simulink model "Simple_EV_Charger"  (R2024b)
settings: Solver=ode8  StartTime=0.0  StopTime=1.5  FixedStep=1e-6  RelTol=1e-3
undefined symbols (not defined in the file): Acid, Lead
libraries: spsDiodeLib x10, spsMosfetLib x6, spsCurrentMeasurementLib x5, spsSeriesRLCBranchLib x5, spsVoltageMeasurementLib x4, slpidlib x3, spsACVoltageSourceLib x1, spsBatteryLib x1, spsLinearTransformerLib x1, spsRMSLib x1, simulink x1, spsIdealSwitchLib x1
settings Model: Creator=SUDHAK1  LastModifiedBy=SUDHAK1

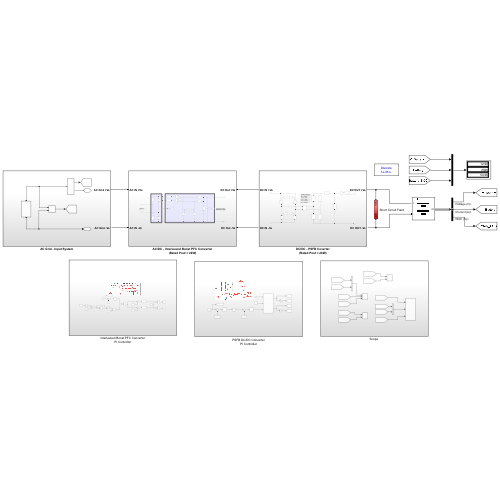
[thumbnail: Simulink's stored preview of the top-level diagram]
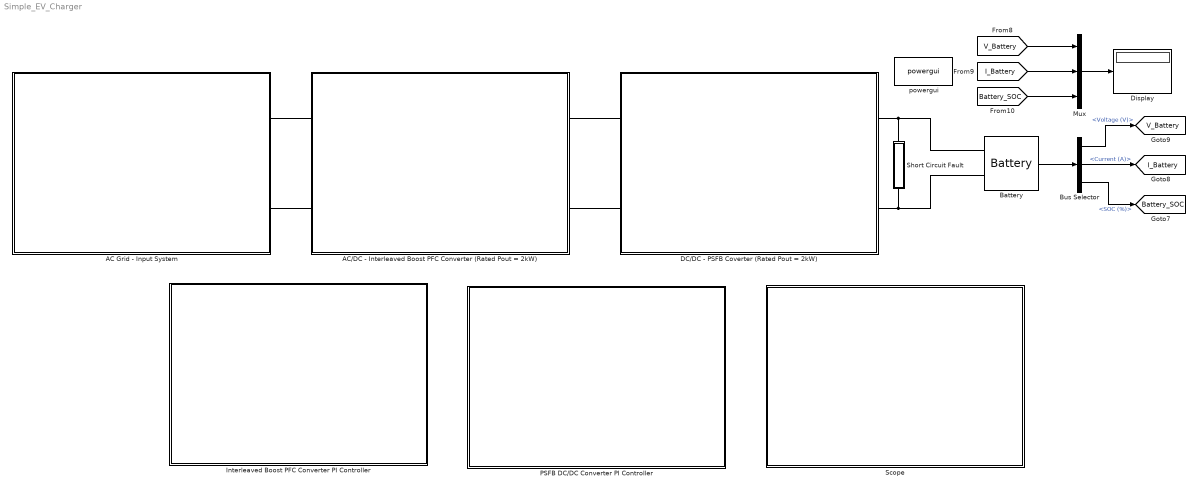
== system Simple_EV_Charger ==
  AC Grid - Input System : Subsystem
  AC/DC - Interleaved Boost PFC Converter (Rated Pout = 2kW) : Subsystem
  Battery : spsBatteryLib/Battery  BatType=Lead-Acid  NomV=48  NomQ=150  SOC=50  Batt_Tr=1  PresetModel=on  MaxQ=156.25  MinV=36  FullV=52.2632  Dis_rate=30  R=0.0032  Normal_OP=46.5417  expZone="[48.8684          0.5]"
  Bus Selector : BusSelector  OutputSignals=Voltage (V),Current (A),SOC (%)
  DC/DC - PSFB Coverter (Rated Pout = 2kW) : Subsystem
  Display : Display
  Interleaved Boost PFC Converter PI Controller : Subsystem
  Mux : Mux  Inputs=3
  PSFB DC/DC Converter PI Controller : Subsystem
  "Scope " : Subsystem
  Short Circuit Fault : Subsystem
      settings: PortSchema="{\"entries\":[{\"content\":{\"sides\":[{\"content\":{},\"type\":\"ConnectorPlacement.EquallySpacedRectSide\",\"uuid\":\"d1eece8f-50e0-4bd3-bd02-64a44f95c15f\"},{\"content\":{\"side\":\"RIGHT\"},\"type\":\"ConnectorPlacement.EquallySpacedRectSide\",\"uuid\":\"d3715762-f460-4a18-a379-b690b190937e\"},{\"content\":{\"connectorIds\":[\"LConn1\"],\"side\":\"TOP\"},\"type\":\"ConnectorPlacement.EquallySpacedRectSide\",\"uuid\":\"cdaaabb7-d644-4e36-8adb-959b7298db19\"},{\"content\":{\"connectorIds\":[\"RConn1\"],\"side\":\"BOTTOM\"},\"type\":\"ConnectorPlacement.EquallySpacedRectSide\",\"uuid\":\"a0244b95-e79a-4abc-836f-bd8cb9c3c8a7\"}]},\"type\":\"ConnectorPlacement.EquallySpacedConnector\",\"uuid\":\"f19808b0-397b-4bab-947c-d2711a911d87\"}],\"packageUris\":[\"http://schema.mathworks.com/mf0/Connector/R2020b\"],\"version\":\"1.0\"}"
  powergui : spspowerguiLib/powergui  Priority=1  SimulationMode=Discrete  SampleTime=1e-6  frequency=60  Iterations=50  frequencyindice=50  Pbase=100e6  ErrMax=1e-4  UnitsV=kV  UnitsW=MW  buscounter=0  FunctionMessages=off  echomessages=off  EnableUseOfTLC=off  CurrentSourceSwitches=off  DisableSnubberDevices=off  DisableRonSwitches=off  DisableVfSwitches=off  DisplayEquations=off  AutomaticDiscreteSolvers=off  SolverType=Tustin/Backward Euler (TBE)  Interpol=off  ExternalGateDelay=off  methode=off  Ts=100  x0status=blocks  SPID=on  SwTol=0  HookPort=off  NonlinearTolerance=1e-4  nMaxIteration=100  ContinueOnMaxIteration=off  RestoreLinks=warning  ResistiveCurrentMeasurement=off  Frange=[0:2:500]  Ylog=off  Xlog=on  ShowGrid=off  save=off  variable=ZData  structure=0  ZoomFFT=off  StartTime=0.0  cycles=1  DisplayStyle=1  fundamental=60  FreqAxis=off  MaxFrequency=1000  frequencyindicesteady=1  RmsSteady=1  display=off
  tag scope: Battery_SOC=global, I_Battery=global, V_Battery=global
  wires:
  Battery/1 -> Bus Selector/1
  Bus Selector/3 -> [Battery_SOC]  "<SOC (%)>"
  Bus Selector/2 -> [I_Battery]  "<Current (A)>"
  Bus Selector/1 -> [V_Battery]  "<Voltage (V)>"
  [V_Battery] -> Mux/1
  [I_Battery] -> Mux/2
  Mux/1 -> Display/1
  [Battery_SOC] -> Mux/3
  connections:
  AC Grid - Input System/RConn1 -- AC/DC - Interleaved Boost PFC Converter (Rated Pout = 2kW)/LConn1
  AC Grid - Input System/RConn2 -- AC/DC - Interleaved Boost PFC Converter (Rated Pout = 2kW)/LConn2
  AC/DC - Interleaved Boost PFC Converter (Rated Pout = 2kW)/RConn1 -- DC/DC - PSFB Coverter (Rated Pout = 2kW)/LConn1
  Battery/LConn1 -- DC/DC - PSFB Coverter (Rated Pout = 2kW)/RConn1 -- Short Circuit Fault/LConn1
  DC/DC - PSFB Coverter (Rated Pout = 2kW)/RConn2 -- Battery/LConn2 -- Short Circuit Fault/RConn1
  DC/DC - PSFB Coverter (Rated Pout = 2kW)/LConn2 -- AC/DC - Interleaved Boost PFC Converter (Rated Pout = 2kW)/RConn2

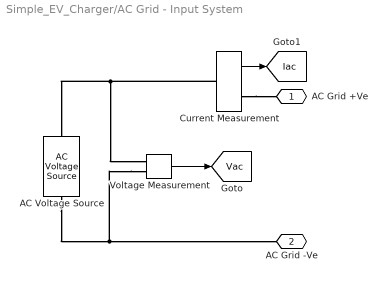
== system Simple_EV_Charger/AC Grid - Input System ==
  AC Voltage Source : spsACVoltageSourceLib/AC Voltage Source  Amplitude=230*sqrt(2)  Phase=0  Frequency=50  SampleTime=0  Measurements=None  BusType=swing  Pref=10e3  Qref=0  Qmin=-inf  Qmax=+inf
  Current Measurement : spsCurrentMeasurementLib/Current Measurement  PhasorSimulation=off  OutputType=Complex  PSBequivalent=0
  Voltage Measurement : spsVoltageMeasurementLib/Voltage Measurement  PhasorSimulation=off  OutputType=Complex  PSBequivalent=0
  AC Grid +Ve : PMIOPort  Side=Right
  AC Grid -Ve : PMIOPort  Port=2  Side=Right
  tag scope: Iac=global, Vac=global
  wires:
  Current Measurement/1 -> [Iac]
  Voltage Measurement/1 -> [Vac]
  connections:
  Voltage Measurement/LConn2 -- AC Grid -Ve/RConn1 -- AC Voltage Source/LConn1
  Current Measurement/LConn1 -- AC Voltage Source/RConn1 -- Voltage Measurement/LConn1
  Current Measurement/RConn1 -- AC Grid +Ve/RConn1

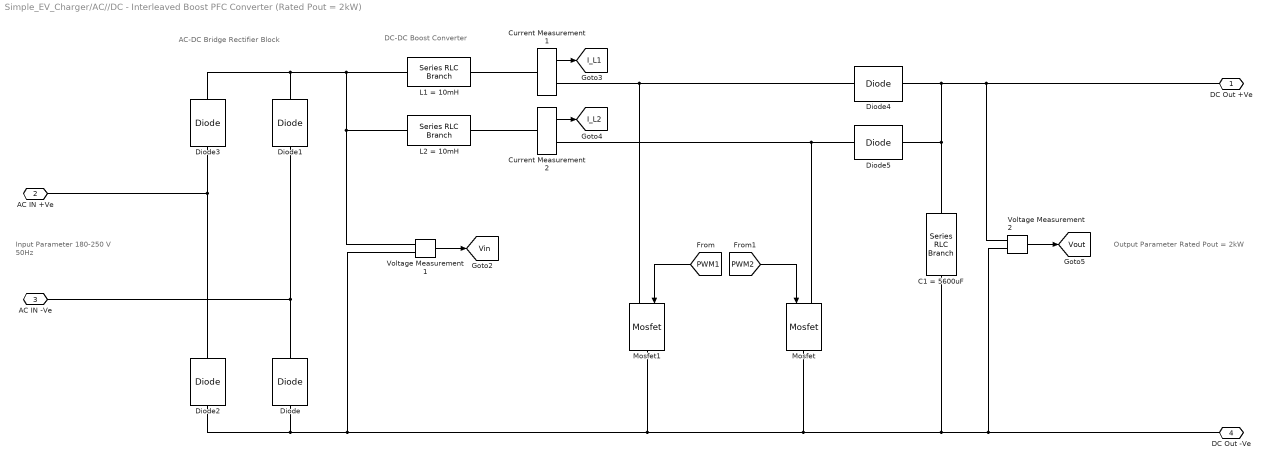
== system Simple_EV_Charger/AC//DC - Interleaved Boost PFC Converter (Rated Pout = 2kW) ==
  note: DC-DC Boost Converter
  note: AC-DC Bridge Rectifier Block
  note: Input Parameter
      | 180-250 V
      | 50Hz
  note: Output Parameter
      | Rated Pout = 2kW
  C1 = 5600uF : spsSeriesRLCBranchLib/Series RLC Branch  LConnTagsString=__new0  RConnTagsString=__new0  BranchType=RC  Resistance=0.02  Inductance=10e-3  SetiL0=off  InitialCurrent=0  Capacitance=5600e-6  Setx0=off  InitialVoltage=0  Measurements=None
  Current Measurement1 : spsCurrentMeasurementLib/Current Measurement  PhasorSimulation=off  OutputType=Complex  PSBequivalent=0
  Current Measurement2 : spsCurrentMeasurementLib/Current Measurement  PhasorSimulation=off  OutputType=Complex  PSBequivalent=0
  Diode{,1..5} (6 alike) : spsDiodeLib/Diode  Ron=1e-3  Lon=0  Vf=0.8  IC=0  UseSnubber=0  Rs=500  Cs=250e-9  Measurements=off
  L1 = 10mH : spsSeriesRLCBranchLib/Series RLC Branch  LConnTagsString=__new0  RConnTagsString=__new0  BranchType=L  Resistance=1  Inductance=10e-3  SetiL0=off  InitialCurrent=0  Capacitance=1e-6  Setx0=off  InitialVoltage=0  Measurements=None
  L2 = 10mH : spsSeriesRLCBranchLib/Series RLC Branch  LConnTagsString=__new0  RConnTagsString=__new0  BranchType=L  Resistance=1  Inductance=10e-3  SetiL0=off  InitialCurrent=0  Capacitance=1e-6  Setx0=off  InitialVoltage=0  Measurements=None
  Mosfet : spsMosfetLib/Mosfet  Ron=0.1  Lon=0  Rd=0.01  Vfd=0  IC=0  Rs=1e5  Cs=inf  Measurements=off
  Mosfet1 : spsMosfetLib/Mosfet  Ron=0.1  Lon=0  Rd=0.01  Vfd=0  IC=0  Rs=1e5  Cs=inf  Measurements=off
  Voltage Measurement1 : spsVoltageMeasurementLib/Voltage Measurement  PhasorSimulation=off  OutputType=Complex  PSBequivalent=0
  Voltage Measurement2 : spsVoltageMeasurementLib/Voltage Measurement  PhasorSimulation=off  OutputType=Complex  PSBequivalent=0
  DC Out +Ve : PMIOPort  Side=Right
  AC IN +Ve : PMIOPort  Port=2  Side=Left
  AC IN -Ve : PMIOPort  Port=3  Side=Left
  DC Out -Ve : PMIOPort  Port=4  Side=Right
  tag scope: I_L1=global, I_L2=global, Vin=global, Vout=global
  wires:
  Current Measurement2/1 -> [I_L2]
  Voltage Measurement2/1 -> [Vout]
  Current Measurement1/1 -> [I_L1]
  Voltage Measurement1/1 -> [Vin]
  [PWM1] -> Mosfet1/1
  [PWM2] -> Mosfet/1
  connections:
  Diode4/LConn1 -- Current Measurement1/RConn1 -- Mosfet1/LConn1
  Diode5/RConn1 -- Diode4/RConn1 -- Voltage Measurement2/LConn1 -- DC Out +Ve/RConn1 -- C1 = 5600uF/LConn1
  Diode5/LConn1 -- Mosfet/LConn1 -- Current Measurement2/RConn1
  Diode1/RConn1 -- L2 = 10mH/LConn1 -- Voltage Measurement1/LConn1 -- L1 = 10mH/LConn1 -- Diode3/RConn1
  Diode2/RConn1 -- AC IN +Ve/RConn1 -- Diode3/LConn1
  Diode/LConn1 -- Voltage Measurement2/LConn2 -- DC Out -Ve/RConn1 -- C1 = 5600uF/RConn1 -- Mosfet/RConn1 -- Mosfet1/RConn1 -- Voltage Measurement1/LConn2 -- Diode2/LConn1
  Diode/RConn1 -- AC IN -Ve/RConn1 -- Diode1/LConn1
  L2 = 10mH/RConn1 -- Current Measurement2/LConn1
  L1 = 10mH/RConn1 -- Current Measurement1/LConn1

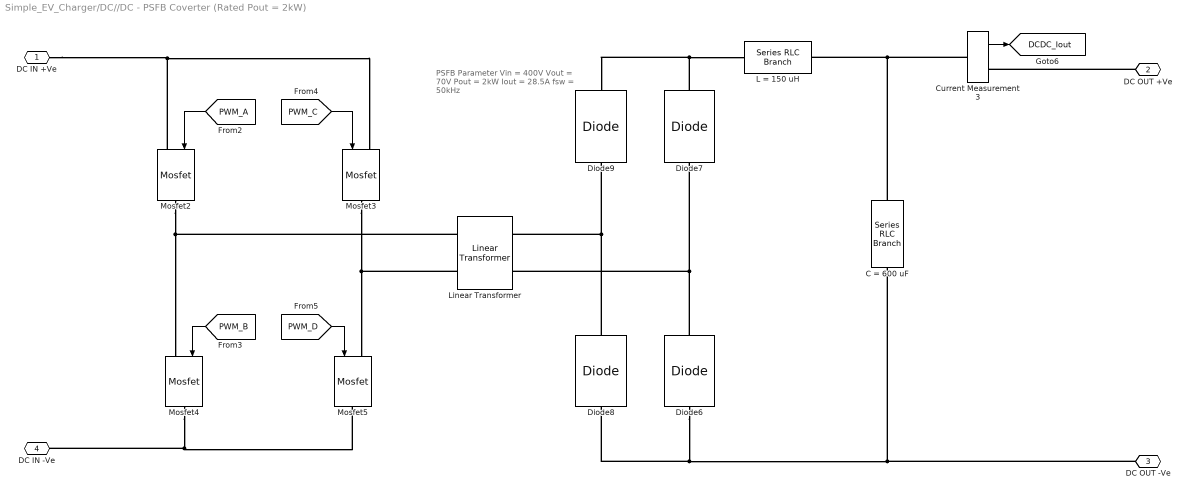
== system Simple_EV_Charger/DC//DC - PSFB Coverter (Rated Pout = 2kW) ==
  note: PSFB Parameter
      | Vin = 400V
      | Vout = 70V
      | Pout = 2kW
      | Iout = 28.5A
      | fsw = 50kHz
  C = 600 uF : spsSeriesRLCBranchLib/Series RLC Branch  LConnTagsString=__new0  RConnTagsString=__new0  BranchType=RC  Resistance=0.02  Inductance=10e-3  SetiL0=off  InitialCurrent=0  Capacitance=600e-6  Setx0=off  InitialVoltage=0  Measurements=None
  Current Measurement3 : spsCurrentMeasurementLib/Current Measurement  PhasorSimulation=off  OutputType=Complex  PSBequivalent=0
  Diode{6..9} (4 alike) : spsDiodeLib/Diode  Ron=1e-6  Lon=0  Vf=0.8  IC=0  UseSnubber=0  Rs=500  Cs=250e-9  Measurements=off
  L = 150 uH : spsSeriesRLCBranchLib/Series RLC Branch  LConnTagsString=__new0  RConnTagsString=__new0  BranchType=L  Resistance=0.02  Inductance=150e-6  SetiL0=off  InitialCurrent=0  Capacitance=5600e-6  Setx0=off  InitialVoltage=0  Measurements=None
  Linear Transformer : spsLinearTransformerLib/Linear Transformer  UNITS=SI  NominalPower=[2000 50e3]  winding1=[400 4.321e-9 0.45586e-9]  winding2=[70 0.7938e-9 0.084225e-9]  ThreeWindings=off  winding3=[3.15e+05 99225 12634]  RmLm=[1.0804e+06 2566]  Measurements=None  DataType=on
  Mosfet{2..5} (4 alike) : spsMosfetLib/Mosfet  Ron=0.1  Lon=0  Rd=0.01  Vfd=0  IC=0  Rs=1e5  Cs=inf  Measurements=off
  DC IN +Ve : PMIOPort  Side=Left
  DC OUT +Ve : PMIOPort  Port=2  Side=Right
  DC OUT -Ve : PMIOPort  Port=3  Side=Right
  DC IN -Ve : PMIOPort  Port=4  Side=Left
  tag scope: DCDC_Iout=global
  wires:
  [PWM_B] -> Mosfet4/1
  [PWM_C] -> Mosfet3/1
  [PWM_D] -> Mosfet5/1
  [PWM_A] -> Mosfet2/1
  Current Measurement3/1 -> [DCDC_Iout]
  connections:
  Diode6/LConn1 -- C = 600 uF/RConn1 -- DC OUT -Ve/RConn1 -- Diode8/LConn1
  Mosfet2/LConn1 -- DC IN +Ve/RConn1 -- Mosfet3/LConn1
  Mosfet2/RConn1 -- Mosfet4/LConn1 -- Linear Transformer/LConn1
  C = 600 uF/LConn1 -- Current Measurement3/LConn1 -- L = 150 uH/RConn1
  Diode8/RConn1 -- Diode9/LConn1 -- Linear Transformer/RConn1
  Mosfet4/RConn1 -- Mosfet5/RConn1 -- DC IN -Ve/RConn1
  Diode6/RConn1 -- Diode7/LConn1 -- Linear Transformer/RConn2
  Diode7/RConn1 -- Diode9/RConn1 -- L = 150 uH/LConn1
  Mosfet3/RConn1 -- Mosfet5/LConn1 -- Linear Transformer/LConn2
  DC OUT +Ve/RConn1 -- Current Measurement3/RConn1

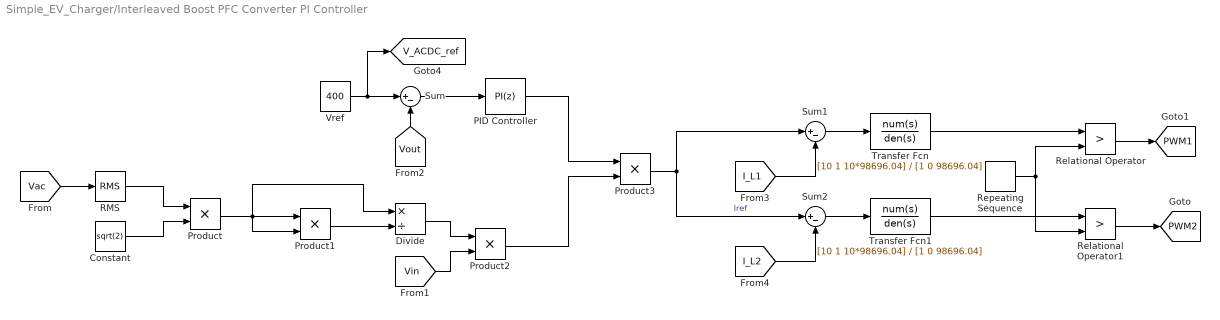
== system Simple_EV_Charger/Interleaved Boost PFC Converter PI Controller ==
  Constant : Constant  Value=sqrt(2)
  Divide : Product  Inputs=*/
  PID Controller : slpidlib/PID Controller  Controller=PI  Form=Parallel  TimeDomain=Discrete-time  UseExternalTs=off  SampleTime=-1  IntegratorMethod=Forward Euler  FilterMethod=Forward Euler  ControllerParametersSource=internal  P=0.25  I=30  UseKiTs=off  D=0  UseExternalDerivativeSource=off  N=100  UseFilter=on  TunerSelectOption=Transfer Function Based (PID Tuner App)  InitialConditionSource=internal  InitialConditionForIntegrator=0  InitialConditionForFilter=0  DifferentiatorICPrevScaledInput=0  ExternalReset=none  TrackingMode=off  Kt=1  LimitOutput=off  SatLimitsSource=internal  UpperSaturationLimit=inf  LowerSaturationLimit=-inf  LinearizeAsGain=on  AntiWindupMode=none  Kb=1  LimitIntegrator=off  UpperIntegratorSaturationLimit=inf  LowerIntegratorSaturationLimit=-inf  POutMin=[]  POutMax=[]  IOutMin=[]  IOutMax=[]  DOutMin=[]  DOutMax=[]  NOutMin=[]  NOutMax=[]  SumOutMin=[]  SumOutMax=[]  SaturationOutMin=[]  SaturationOutMax=[]  PParamMin=[]  PParamMax=[]  IParamMin=[]  IParamMax=[]  DParamMin=[]  DParamMax=[]  NParamMin=[]  NParamMax=[]  KbParamMin=[]  KbParamMax=[]  KtParamMin=[]  KtParamMax=[]  KbOutMin=[]  KbOutMax=[]  KtOutMin=[]  KtOutMax=[]  IntegratorOutMin=[]  IntegratorOutMax=[]  FilterOutMin=[]  FilterOutMax=[]  SumI1OutMin=[]  SumI1OutMax=[]  SumI2OutMin=[]  SumI2OutMax=[]  SumI3OutMin=[]  SumI3OutMax=[]  SumI4OutMin=[]  SumI4OutMax=[]  SumDOutMin=[]  SumDOutMax=[]  DifferentiatorOutMin=[]  DifferentiatorOutMax=[]  FilterDiffOutCoefMin=[]  FilterDiffOutCoefMax=[]  ReciprocalOutMin=[]  ReciprocalOutMax=[]  SumDenOutMin=[]  SumDenOutMax=[]  SumNumOutMin=[]  SumNumOutMax=[]  DivideOutMin=[]  DivideOutMax=[]  UdiffTsProdOutMin=[]  UdiffTsProdOutMax=[]  NTsProdOutMin=[]  NTsProdOutMax=[]  UintegralTsProdOutMin=[]  UintegralTsProdOutMax=[]  UngainTsProdOutMin=[]  UngainTsProdOutMax=[]  ClampingZeroOutDataTypeStr=Inherit: Inherit via back propagation  ClampingZeroOutMin=[]  ClampingZeroOutMax=[]  FilterDenConstantOutDataTypeStr=Inherit: Inherit via back propagation  FilterDenConstantOutMin=[]  FilterDenConstantOutMax=[]  PCopyOutDataTypeStr=Inherit: Inherit via back propagation  PCopyOutMin=[]  PCopyOutMax=[]  NCopyOutDataTypeStr=Inherit: Inherit via back propagation  NCopyOutMin=[]  NCopyOutMax=[]  IntegratorContinuousStateAttributes=''  IntegratorStateMustResolveToSignalObject=off  IntegratorRTWStateStorageClass=Auto  FilterContinuousStateAttributes=''  FilterStateMustResolveToSignalObject=off  FilterRTWStateStorageClass=Auto  ParallelPVariant=InternalParameters  IdealPVariant=Disabled  IVariant=InternalParameters  DVariant=Disabled  IntegratorVariant=Discrete  SatVariant=Disabled  AWVariant=Passthrough  PCopyVariant=Disabled  TRVariant=Disabled  FdbkBlocksVariant=Forward  IdealPFdbkVariant=Disabled  SatFdbkVariant=Disabled  DerivativeFilterVariant=Disabled  NVariant=Disabled  NCopyVariant=Disabled_SignalSpec  FilterICVariant=Disabled  IntegratorICVariant=InternalICs  ExternalResetVariant=Disabled  TRSumVariant=Passthrough  SumFdbkVariant=Disabled  SumVariant=Sum_PI  TsampFilterVariant=InternalTs  TsampNgainVariant=Passthrough  TsampIntegralVariant=Disabled_SignalSpec  ExternalSaturationOutDataTypeStr=Inherit: Same as second input  DerivativeSourceVariant=Disabled  PreIntVariant=InternalPreInt
  Product{,1..3} (4 alike) : Product
  RMS : spsRMSLib/RMS  TrueRMS=on  Freq=50  RMSInit=230  Ts=0
  Relational Operator : RelationalOperator  Operator=>  OutDataTypeStr=boolean  RndMeth=Simplest  InputSameDT=off
  Relational Operator1 : RelationalOperator  Operator=>  OutDataTypeStr=boolean  RndMeth=Simplest  InputSameDT=off
  Repeating Sequence : simulink/Sources/Repeating Sequence  rep_seq_t=[0 1/10000 1/5000]  rep_seq_y=[0 1 0]
  Sum : Sum  Inputs=|+-
  Sum1 : Sum  Inputs=|+-
  Sum2 : Sum  Inputs=|+-
  Transfer Fcn : TransferFcn  Numerator=[10 1 10*98696.04]  Denominator=[1 0 98696.04]
  Transfer Fcn1 : TransferFcn  Numerator=[10 1 10*98696.04]  Denominator=[1 0 98696.04]
  Vref : Constant  Value=400
  tag scope: PWM1=global, PWM2=global, V_ACDC_ref=global
  wires:
  Constant/1 -> Product/2
  Product/1 -> Product1/1, Divide/1, Product1/2
  Product1/1 -> Divide/2
  [Vac] -> RMS/1
  RMS/1 -> Product/1
  [Vin] -> Product2/2
  Divide/1 -> Product2/1
  Vref/1 -> [V_ACDC_ref], Sum/1
  [Vout] -> Sum/2
  Sum/1 -> PID Controller/1
  PID Controller/1 -> Product3/1
  Product2/1 -> Product3/2
  Product3/1 -> Sum2/1, Sum1/1  "Iref"
  [I_L1] -> Sum1/2
  [I_L2] -> Sum2/2
  Sum1/1 -> Transfer Fcn/1
  Sum2/1 -> Transfer Fcn1/1
  Transfer Fcn/1 -> Relational Operator/1
  Repeating Sequence/1 -> Relational Operator1/2, Relational Operator/2
  Transfer Fcn1/1 -> Relational Operator1/1
  Relational Operator1/1 -> [PWM2]
  Relational Operator/1 -> [PWM1]

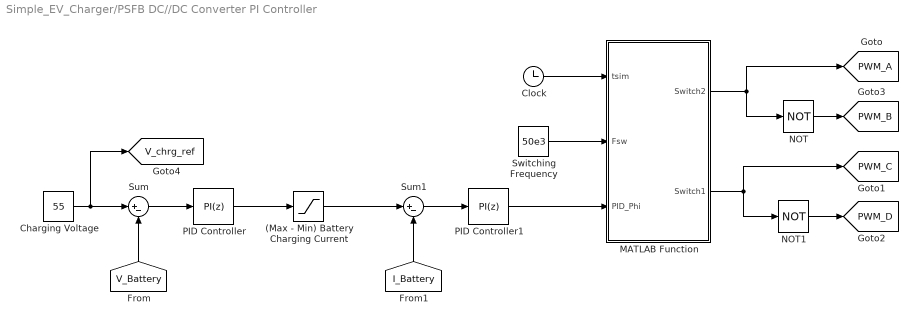
== system Simple_EV_Charger/PSFB DC//DC Converter PI Controller ==
  (Max - Min) Battery Charging Current : Saturate  UpperLimit=37.5  LowerLimit=0
  Charging Voltage : Constant  Value=55
  Clock : Clock
  MATLAB Function : MATLAB Function  TreatAsAtomicUnit=on
  NOT : Logic  Operator=NOT  IconShape=distinctive  AllPortsSameDT=off  OutDataTypeStr=boolean
  NOT1 : Logic  Operator=NOT  IconShape=distinctive  AllPortsSameDT=off  OutDataTypeStr=boolean
  PID Controller : slpidlib/PID Controller  Controller=PI  Form=Parallel  TimeDomain=Discrete-time  UseExternalTs=off  SampleTime=-1  IntegratorMethod=Forward Euler  FilterMethod=Forward Euler  ControllerParametersSource=internal  P=25  I=5  UseKiTs=off  D=0  UseExternalDerivativeSource=off  N=100  UseFilter=on  TunerSelectOption=Transfer Function Based (PID Tuner App)  InitialConditionSource=internal  InitialConditionForIntegrator=0  InitialConditionForFilter=0  DifferentiatorICPrevScaledInput=0  ExternalReset=none  TrackingMode=off  Kt=1  LimitOutput=on  SatLimitsSource=internal  UpperSaturationLimit=180  LowerSaturationLimit=0  LinearizeAsGain=on  AntiWindupMode=none  Kb=1  LimitIntegrator=off  UpperIntegratorSaturationLimit=70  LowerIntegratorSaturationLimit=0  POutMin=[]  POutMax=[]  IOutMin=[]  IOutMax=[]  DOutMin=[]  DOutMax=[]  NOutMin=[]  NOutMax=[]  SumOutMin=[]  SumOutMax=[]  SaturationOutMin=[]  SaturationOutMax=[]  PParamMin=[]  PParamMax=[]  IParamMin=[]  IParamMax=[]  DParamMin=[]  DParamMax=[]  NParamMin=[]  NParamMax=[]  KbParamMin=[]  KbParamMax=[]  KtParamMin=[]  KtParamMax=[]  KbOutMin=[]  KbOutMax=[]  KtOutMin=[]  KtOutMax=[]  IntegratorOutMin=[]  IntegratorOutMax=[]  FilterOutMin=[]  FilterOutMax=[]  SumI1OutMin=[]  SumI1OutMax=[]  SumI2OutMin=[]  SumI2OutMax=[]  SumI3OutMin=[]  SumI3OutMax=[]  SumI4OutMin=[]  SumI4OutMax=[]  SumDOutMin=[]  SumDOutMax=[]  DifferentiatorOutMin=[]  DifferentiatorOutMax=[]  FilterDiffOutCoefMin=[]  FilterDiffOutCoefMax=[]  ReciprocalOutMin=[]  ReciprocalOutMax=[]  SumDenOutMin=[]  SumDenOutMax=[]  SumNumOutMin=[]  SumNumOutMax=[]  DivideOutMin=[]  DivideOutMax=[]  UdiffTsProdOutMin=[]  UdiffTsProdOutMax=[]  NTsProdOutMin=[]  NTsProdOutMax=[]  UintegralTsProdOutMin=[]  UintegralTsProdOutMax=[]  UngainTsProdOutMin=[]  UngainTsProdOutMax=[]  ClampingZeroOutDataTypeStr=Inherit: Inherit via back propagation  ClampingZeroOutMin=[]  ClampingZeroOutMax=[]  FilterDenConstantOutDataTypeStr=Inherit: Inherit via back propagation  FilterDenConstantOutMin=[]  FilterDenConstantOutMax=[]  PCopyOutDataTypeStr=Inherit: Inherit via back propagation  PCopyOutMin=[]  PCopyOutMax=[]  NCopyOutDataTypeStr=Inherit: Inherit via back propagation  NCopyOutMin=[]  NCopyOutMax=[]  IntegratorContinuousStateAttributes=''  IntegratorStateMustResolveToSignalObject=off  IntegratorRTWStateStorageClass=Auto  FilterContinuousStateAttributes=''  FilterStateMustResolveToSignalObject=off  FilterRTWStateStorageClass=Auto  ParallelPVariant=InternalParameters  IdealPVariant=Disabled  IVariant=InternalParameters  DVariant=Disabled  IntegratorVariant=Discrete  SatVariant=Enabled  AWVariant=Passthrough  PCopyVariant=Disabled  TRVariant=Disabled  FdbkBlocksVariant=Forward  IdealPFdbkVariant=Disabled  SatFdbkVariant=Disabled  DerivativeFilterVariant=Disabled  NVariant=Disabled  NCopyVariant=Disabled_SignalSpec  FilterICVariant=Disabled  IntegratorICVariant=InternalICs  ExternalResetVariant=Disabled  TRSumVariant=Passthrough  SumFdbkVariant=Disabled  SumVariant=Sum_PI  TsampFilterVariant=InternalTs  TsampNgainVariant=Passthrough  TsampIntegralVariant=Disabled_SignalSpec  ExternalSaturationOutDataTypeStr=Inherit: Same as second input  DerivativeSourceVariant=Disabled  PreIntVariant=InternalPreInt
  PID Controller1 : slpidlib/PID Controller  Controller=PI  Form=Parallel  TimeDomain=Discrete-time  UseExternalTs=off  SampleTime=-1  IntegratorMethod=Forward Euler  FilterMethod=Forward Euler  ControllerParametersSource=internal  P=25  I=5  UseKiTs=off  D=0  UseExternalDerivativeSource=off  N=100  UseFilter=on  TunerSelectOption=Transfer Function Based (PID Tuner App)  InitialConditionSource=internal  InitialConditionForIntegrator=0  InitialConditionForFilter=0  DifferentiatorICPrevScaledInput=0  ExternalReset=none  TrackingMode=off  Kt=1  LimitOutput=on  SatLimitsSource=internal  UpperSaturationLimit=180  LowerSaturationLimit=0  LinearizeAsGain=on  AntiWindupMode=none  Kb=1  LimitIntegrator=off  UpperIntegratorSaturationLimit=70  LowerIntegratorSaturationLimit=0  POutMin=[]  POutMax=[]  IOutMin=[]  IOutMax=[]  DOutMin=[]  DOutMax=[]  NOutMin=[]  NOutMax=[]  SumOutMin=[]  SumOutMax=[]  SaturationOutMin=[]  SaturationOutMax=[]  PParamMin=[]  PParamMax=[]  IParamMin=[]  IParamMax=[]  DParamMin=[]  DParamMax=[]  NParamMin=[]  NParamMax=[]  KbParamMin=[]  KbParamMax=[]  KtParamMin=[]  KtParamMax=[]  KbOutMin=[]  KbOutMax=[]  KtOutMin=[]  KtOutMax=[]  IntegratorOutMin=[]  IntegratorOutMax=[]  FilterOutMin=[]  FilterOutMax=[]  SumI1OutMin=[]  SumI1OutMax=[]  SumI2OutMin=[]  SumI2OutMax=[]  SumI3OutMin=[]  SumI3OutMax=[]  SumI4OutMin=[]  SumI4OutMax=[]  SumDOutMin=[]  SumDOutMax=[]  DifferentiatorOutMin=[]  DifferentiatorOutMax=[]  FilterDiffOutCoefMin=[]  FilterDiffOutCoefMax=[]  ReciprocalOutMin=[]  ReciprocalOutMax=[]  SumDenOutMin=[]  SumDenOutMax=[]  SumNumOutMin=[]  SumNumOutMax=[]  DivideOutMin=[]  DivideOutMax=[]  UdiffTsProdOutMin=[]  UdiffTsProdOutMax=[]  NTsProdOutMin=[]  NTsProdOutMax=[]  UintegralTsProdOutMin=[]  UintegralTsProdOutMax=[]  UngainTsProdOutMin=[]  UngainTsProdOutMax=[]  ClampingZeroOutDataTypeStr=Inherit: Inherit via back propagation  ClampingZeroOutMin=[]  ClampingZeroOutMax=[]  FilterDenConstantOutDataTypeStr=Inherit: Inherit via back propagation  FilterDenConstantOutMin=[]  FilterDenConstantOutMax=[]  PCopyOutDataTypeStr=Inherit: Inherit via back propagation  PCopyOutMin=[]  PCopyOutMax=[]  NCopyOutDataTypeStr=Inherit: Inherit via back propagation  NCopyOutMin=[]  NCopyOutMax=[]  IntegratorContinuousStateAttributes=''  IntegratorStateMustResolveToSignalObject=off  IntegratorRTWStateStorageClass=Auto  FilterContinuousStateAttributes=''  FilterStateMustResolveToSignalObject=off  FilterRTWStateStorageClass=Auto  ParallelPVariant=InternalParameters  IdealPVariant=Disabled  IVariant=InternalParameters  DVariant=Disabled  IntegratorVariant=Discrete  SatVariant=Enabled  AWVariant=Passthrough  PCopyVariant=Disabled  TRVariant=Disabled  FdbkBlocksVariant=Forward  IdealPFdbkVariant=Disabled  SatFdbkVariant=Disabled  DerivativeFilterVariant=Disabled  NVariant=Disabled  NCopyVariant=Disabled_SignalSpec  FilterICVariant=Disabled  IntegratorICVariant=InternalICs  ExternalResetVariant=Disabled  TRSumVariant=Passthrough  SumFdbkVariant=Disabled  SumVariant=Sum_PI  TsampFilterVariant=InternalTs  TsampNgainVariant=Passthrough  TsampIntegralVariant=Disabled_SignalSpec  ExternalSaturationOutDataTypeStr=Inherit: Same as second input  DerivativeSourceVariant=Disabled  PreIntVariant=InternalPreInt
  Sum : Sum  Inputs=|+-
  Sum1 : Sum  Inputs=|+-
  Switching Frequency : Constant  Value=50e3
  tag scope: PWM_A=global, PWM_B=global, PWM_C=global, PWM_D=global, V_chrg_ref=global
  wires:
  Charging Voltage/1 -> [V_chrg_ref], Sum/1
  [V_Battery] -> Sum/2
  Sum/1 -> PID Controller/1
  PID Controller/1 -> (Max - Min) Battery Charging Current/1
  (Max - Min) Battery Charging Current/1 -> Sum1/1
  [I_Battery] -> Sum1/2
  Sum1/1 -> PID Controller1/1
  PID Controller1/1 -> MATLAB Function/3(PID_Phi)
  Switching Frequency/1 -> MATLAB Function/2(Fsw)
  Clock/1 -> MATLAB Function/1(tsim)
  NOT/1 -> [PWM_B]
  MATLAB Function/1(Switch2) -> [PWM_A], NOT/1
  NOT1/1 -> [PWM_D]
  MATLAB Function/2(Switch1) -> [PWM_C], NOT1/1

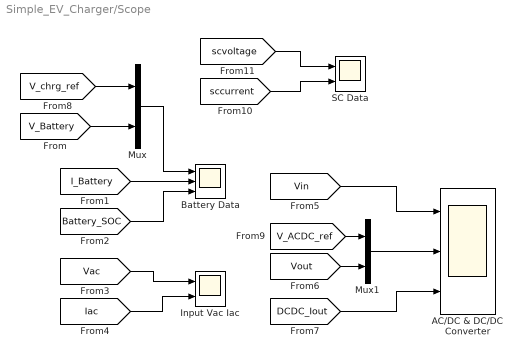
== system Simple_EV_Charger/Scope  ==
  AC/DC & DC/DC Converter : Scope  NumInputPorts=3
  Battery Data : Scope  NumInputPorts=3
  Input Vac Iac : Scope  NumInputPorts=2
  Mux : Mux  Inputs=2
  Mux1 : Mux  Inputs=2
  SC Data : Scope  NumInputPorts=2
  wires:
  [Iac] -> Input Vac Iac/2
  [Vout] -> Mux1/2
  [Battery_SOC] -> Battery Data/3
  [Vac] -> Input Vac Iac/1
  [DCDC_Iout] -> AC/DC & DC/DC Converter/3
  [V_Battery] -> Mux/2
  [Vin] -> AC/DC & DC/DC Converter/1
  [I_Battery] -> Battery Data/2
  [V_chrg_ref] -> Mux/1
  Mux/1 -> Battery Data/1
  [V_ACDC_ref] -> Mux1/1
  Mux1/1 -> AC/DC & DC/DC Converter/2
  [sccurrent] -> SC Data/2
  [scvoltage] -> SC Data/1

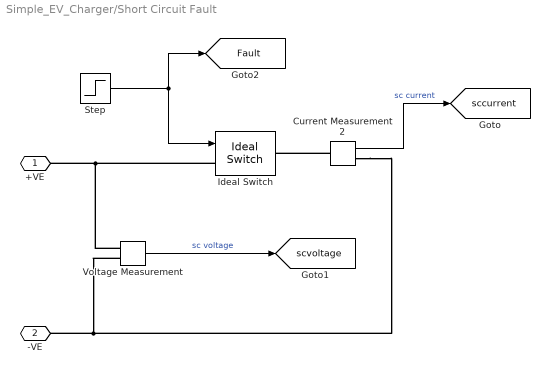
== system Simple_EV_Charger/Short Circuit Fault ==
  Current Measurement2 : spsCurrentMeasurementLib/Current Measurement  PhasorSimulation=off  OutputType=Complex  PSBequivalent=0
  Ideal Switch : spsIdealSwitchLib/Ideal Switch  Ron=5e-3  Lon=0  IC=0  Rs=1e5  Cs=inf  Measurements=off
  Step : Step  Time=0.5  SampleTime=0
  Voltage Measurement : spsVoltageMeasurementLib/Voltage Measurement  PhasorSimulation=off  OutputType=Complex  PSBequivalent=0
  +VE : PMIOPort  Side=Left
  -VE : PMIOPort  Port=2  Side=Right
  tag scope: Fault=global, sccurrent=global, scvoltage=global
  wires:
  Step/1 -> Ideal Switch/1, [Fault]
  Current Measurement2/1 -> [sccurrent]  "sc current"
  Voltage Measurement/1 -> [scvoltage]  "sc voltage"
  connections:
  Current Measurement2/RConn1 -- Voltage Measurement/LConn2 -- -VE/RConn1
  Ideal Switch/LConn1 -- Voltage Measurement/LConn1 -- +VE/RConn1
  Current Measurement2/LConn1 -- Ideal Switch/RConn1

== matlab function Simple_EV_Charger/PSFB DC//DC Converter PI Controller/MATLAB Function ==
  data: tsim input; Switch2 output; Switch1 output; Fsw input; PID_Phi input
function [Switch2,Switch1] = fcn(tsim,Fsw,PID_Phi)

% Inputs
% tsim = simulation time [s]
% Fsw = switching frequency [Hz]
% PID_Phi = Phase Difference or Phase-shift command from the closed-loop PID controller [degrees]

% Outputs
% Switch1 = switching pulse for bridge signal 1
% Switch2 = phase-shifted switching pulse for bridge signal 2

Tsw = 1/Fsw; %Switching time period calculation

Switch2=0;
Switch1=0;

remainder_value_1 = mod(tsim,Tsw);

if remainder_value_1 < Tsw/2 % creates a 50% duty-cycle square wave
    Switch1 = 1;
end

time_delay = Tsw*PID_Phi/360; %converts phase angle in degrees into an equivalent time delay:

remainder_value_2 = mod(tsim+time_delay , Tsw); %generates a waveform shifted relative to Switch1

if remainder_value_2 < Tsw/2 % creates a 50% duty-cycle square wave
    Switch2 = 1;
end
